simulink model "EV6_LUT_FourWheel_EV6Battery77p4kWh_PowerCorrected"  (R2024a)
settings: Solver=ode4  StartTime=0  StopTime=60  FixedStep=0.001  RelTol=1e-3
PreLoadFcn:
  | VSS_BICYCLE=Simulink.Variant('Dual=0');
  | VSS_DUAL=Simulink.Variant('Dual=1');
  | Dual=1;
  | load('DriveCycle2.mat')
PostLoadFcn:
  | if any(exist('dsrtsu_mdlpostloadfcn', 'file') ~= 0), dsrtsu_mdlpostloadfcn('Execute', bdroot); end
InitFcn:
  | , if any(exist('rtifpga_mdlclblib', 'file') ~= 0), rtifpga_mdlclblib('Init', bdroot); end,
  | , if any(exist('dsmpb_private', 'file') ~= 0), dsmpb_private('dsmpb_mdlclblib', 'Init', bdroot); end,
  | load('DriveCycle2.mat')
model workspace (MAT data in the model file):
  DiffRatio = 10.65
  EV6_2023_BattBranchCapacity_Ah = 55.5236728838
  EV6_2023_BattEnergy_kWh = 77.4
  EV6_2023_BattNominalVoltage_V = 697
  EV6_2023_BattNumCellsParallel = 2
  EV6_2023_BattNumCellsSeries = 192
  EV6_2023_BattOpenVoltCapBpts = [0 0.1 0.2 0.3 0.4 0.5 0.6 0.7 0.8 0.9 1]
  EV6_2023_BattOpenVoltTbl = [2.96762142548 3.40364281191 3.47417488548 3.54470541822 3.61523441014 3.68576186124 3.75628777151 3.82681214095 3.94527005036 4.07101207308 4.2120755254]
  EV6_2023_BattPackCapacity_Ah = 111.047345768
  EV6_2023_BattResistSocBpts = [0 0.2 0.4 0.6 0.8 1]
  EV6_2023_BattResistTbl = [0.0163620057716 0.0118174152018 0.00807187352333 0.00375663957972 0.00266904525531 0.00103635901355 0.0019014404175 0.0172368903217 0.0121226074867 0.00758541551769 0.00474065349228 0.00337561163613 ... (42 elements, 7x6)]
  EV6_2023_BattResistTempBpts = [243.1 253.1 263.1 273.1 283.1 298.1 313.1]
  EV6_2023_InitialPackOCV_V = 726.471714233
  EV6_2023_InitialSOC = 0.638878863672
  EV6_BattCellCapacity_Ah = 60.3
  EV6_BattInitialSOC = 0.638878863672
  EV6_BattOCV_Cell_V = [2.96762142548 3.40364281191 3.47417488548 3.54470541822 3.61523441014 3.68576186124 3.75628777151 3.82681214095 3.94527005036 4.07101207308 4.2120755254]
  EV6_BattOCV_SOC = [0 0.1 0.2 0.3 0.4 0.5 0.6 0.7 0.8 0.9 1]
  EV6_BattPackCapacity_Ah = 120.6
  EV6_BattParallelCells = 2
  EV6_BattResistanceSOC = [0 0.2 0.4 0.6 0.8 1]
  EV6_BattResistanceTable_Ohm = [0.0163620057716 0.0118174152018 0.00807187352333 0.00375663957972 0.00266904525531 0.00103635901355 0.0019014404175 0.0172368903217 0.0121226074867 0.00758541551769 0.00474065349228 0.00337561163613 ... (42 elements, 7x6)]
  EV6_BattResistanceTemp_K = [243.1 253.1 263.1 273.1 283.1 298.1 313.1]
  EV6_BattSeriesCells = 192
  EV6_FinalDriveRatio = 10.65
  EV6_TargetPackResistance_Ohm = 0.132763804608
  Gas = 0.383333333333
undefined symbols (not defined in the file): accel_bp_mps2, AccelCmd, ActTqLF_Nm_, ActTqLR_Nm_, ActTqRF_Nm_, ActTqRR_Nm_, BattChargeLimitMaxPwr, BattChargeLimitSocBpts, BattChargeLimitTbl, BattDischargeLimitSocBpts, BattDischargeLimitTbl, BattDischargeMaxPwr, BrakeMaxPrs, BrakeMaxTrq, ChassisDistCg2FrontAxle, ChassisDistCg2RearAxle, ChassisVehMass, CltchCmd, CoastDown, DecelCmd, DiscIntNeverNeededParam, EnvGravCnst, EnvPrs, EnvTemp, EV6_RegenTorqueGain, EV6_TractionTorqueGain, front_share_regen_3d, front_share_traction_3d, FuelSpecificGrav, GearCmd, h, InitStates, lgSw, limitedMCT, MCT, MtrEffSpdBpts, MtrEffTbl, MtrEffTrqBpts, MtrPwrMax, MtrTrqMax, out_1, pMCT, RealSimPara, Ref_speed, Ref_time, regen_torque_bp_Nm, speed_bp_kph, SteeringCmd, SupvsryCtrlRegenBrkCutOffTbl, SupvsryCtrlRegenSpdBpts, TestScnrioCycleNum, traction_torque_bp_Nm, US06, VEH
libraries: VSIGenLib x65, simulink x54, etargetslib x38, dsmpblib x24, vehdynlibtire x12, autolibshared x11, vehdynlibsuspension x7, vehdynlibtirecommon x7, autolibpowerinfoutils x6, autolibutils x5, autolibsharedcoupling x4, autolibmappedmotor x4
(part 3 of 19)

== system EV6_LUT_FourWheel_EV6Battery77p4kWh_PowerCorrected/RealSim1/ToRealSim/RealSim CreatBus ==
  In : Inport
  speedDesired : Inport  Port=2
  color : Inport  Port=3
  accelerationDesired : Inport  Port=4
  activeLaneChange : Inport  Port=5
  Bus Creator2 : BusCreator  Inputs=36  OutDataTypeStr=Bus: VehDataBus
  Bus Selector1 : BusSelector  OutputSignals=id,idLength,type,typeLength,vehicleClass,vehicleClassLength,speed,acceleration,positionX,positionY,positionZ,heading,color,linkId,linkIdLength,laneId,distanceTravel,speedDesired,accelerationDesired,hasPrecedingVehicle,precedingVehicleId,precedingVehicleIdLength,precedingVehicleDistance,precedingVehicleSpeed,signalLightId,signalLightIdLength,signalLightHeadId,signalLightDistance,signalLightColor,speedLimit,speedLimitNext,speedLimitChangeDistance,linkIdNext,linkIdNextLength,grade,activeLaneChange
  Terminator{4..7} (4 alike) : Terminator
  rgba2uint : Subsystem
  Out : Outport
  wires:
  Bus Creator2/1 -> Out/1
  rgba2uint/1(Out1) -> Bus Creator2/13  "color"
  color/1 -> rgba2uint/1(In1)  "color"
  accelerationDesired/1 -> Bus Creator2/19  "accelerationDesired"
  speedDesired/1 -> Bus Creator2/18  "speedDesired"
  activeLaneChange/1 -> Bus Creator2/36  "activeLaneChange"
  Bus Selector1/36 -> Terminator7/1  "<activeLaneChange>"
  Bus Selector1/35 -> Bus Creator2/35  "<grade>"
  Bus Selector1/34 -> Bus Creator2/34  "<linkIdNextLength>"
  Bus Selector1/33 -> Bus Creator2/33  "<linkIdNext>"
  Bus Selector1/32 -> Bus Creator2/32  "<speedLimitChangeDistance>"
  Bus Selector1/31 -> Bus Creator2/31  "<speedLimitNext>"
  Bus Selector1/30 -> Bus Creator2/30  "<speedLimit>"
  Bus Selector1/29 -> Bus Creator2/29  "<signalLightColor>"
  Bus Selector1/28 -> Bus Creator2/28  "<signalLightDistance>"
  Bus Selector1/27 -> Bus Creator2/27  "<signalLightHeadId>"
  Bus Selector1/26 -> Bus Creator2/26  "<signalLightIdLength>"
  Bus Selector1/25 -> Bus Creator2/25  "<signalLightId>"
  Bus Selector1/24 -> Bus Creator2/24  "<precedingVehicleSpeed>"
  Bus Selector1/23 -> Bus Creator2/23  "<precedingVehicleDistance>"
  Bus Selector1/22 -> Bus Creator2/22  "<precedingVehicleIdLength>"
  Bus Selector1/21 -> Bus Creator2/21  "<precedingVehicleId>"
  Bus Selector1/20 -> Bus Creator2/20  "<hasPrecedingVehicle>"
  Bus Selector1/19 -> Terminator6/1  "<accelerationDesired>"
  Bus Selector1/18 -> Terminator4/1  "<speedDesired>"
  Bus Selector1/17 -> Bus Creator2/17  "<distanceTravel>"
  Bus Selector1/16 -> Bus Creator2/16  "<laneId>"
  Bus Selector1/15 -> Bus Creator2/15  "<linkIdLength>"
  Bus Selector1/14 -> Bus Creator2/14  "<linkId>"
  Bus Selector1/13 -> Terminator5/1  "<color>"
  Bus Selector1/12 -> Bus Creator2/12  "<heading>"
  Bus Selector1/11 -> Bus Creator2/11  "<positionZ>"
  Bus Selector1/10 -> Bus Creator2/10  "<positionY>"
  Bus Selector1/9 -> Bus Creator2/9  "<positionX>"
  Bus Selector1/8 -> Bus Creator2/8  "<acceleration>"
  Bus Selector1/7 -> Bus Creator2/7  "<speed>"
  Bus Selector1/6 -> Bus Creator2/6  "<vehicleClassLength>"
  Bus Selector1/5 -> Bus Creator2/5  "<vehicleClass>"
  Bus Selector1/4 -> Bus Creator2/4  "<typeLength>"
  Bus Selector1/3 -> Bus Creator2/3  "<type>"
  Bus Selector1/2 -> Bus Creator2/2  "<idLength>"
  Bus Selector1/1 -> Bus Creator2/1  "<id>"
  In/1 -> Bus Selector1/1

== system EV6_LUT_FourWheel_EV6Battery77p4kWh_PowerCorrected/RealSim2/ToRealSim/RealSim CreatBus ==
  In : Inport
  speedDesired : Inport  Port=2
  color : Inport  Port=3
  accelerationDesired : Inport  Port=4
  activeLaneChange : Inport  Port=5
  Bus Creator2 : BusCreator  Inputs=36  OutDataTypeStr=Bus: VehDataBus
  Bus Selector1 : BusSelector  OutputSignals=id,idLength,type,typeLength,vehicleClass,vehicleClassLength,speed,acceleration,positionX,positionY,positionZ,heading,color,linkId,linkIdLength,laneId,distanceTravel,speedDesired,accelerationDesired,hasPrecedingVehicle,precedingVehicleId,precedingVehicleIdLength,precedingVehicleDistance,precedingVehicleSpeed,signalLightId,signalLightIdLength,signalLightHeadId,signalLightDistance,signalLightColor,speedLimit,speedLimitNext,speedLimitChangeDistance,linkIdNext,linkIdNextLength,grade,activeLaneChange
  Terminator{4..7} (4 alike) : Terminator
  rgba2uint : Subsystem
  Out : Outport
  wires:
  Bus Creator2/1 -> Out/1
  rgba2uint/1(Out1) -> Bus Creator2/13  "color"
  color/1 -> rgba2uint/1(In1)  "color"
  accelerationDesired/1 -> Bus Creator2/19  "accelerationDesired"
  speedDesired/1 -> Bus Creator2/18  "speedDesired"
  activeLaneChange/1 -> Bus Creator2/36  "activeLaneChange"
  Bus Selector1/36 -> Terminator7/1  "<activeLaneChange>"
  Bus Selector1/35 -> Bus Creator2/35  "<grade>"
  Bus Selector1/34 -> Bus Creator2/34  "<linkIdNextLength>"
  Bus Selector1/33 -> Bus Creator2/33  "<linkIdNext>"
  Bus Selector1/32 -> Bus Creator2/32  "<speedLimitChangeDistance>"
  Bus Selector1/31 -> Bus Creator2/31  "<speedLimitNext>"
  Bus Selector1/30 -> Bus Creator2/30  "<speedLimit>"
  Bus Selector1/29 -> Bus Creator2/29  "<signalLightColor>"
  Bus Selector1/28 -> Bus Creator2/28  "<signalLightDistance>"
  Bus Selector1/27 -> Bus Creator2/27  "<signalLightHeadId>"
  Bus Selector1/26 -> Bus Creator2/26  "<signalLightIdLength>"
  Bus Selector1/25 -> Bus Creator2/25  "<signalLightId>"
  Bus Selector1/24 -> Bus Creator2/24  "<precedingVehicleSpeed>"
  Bus Selector1/23 -> Bus Creator2/23  "<precedingVehicleDistance>"
  Bus Selector1/22 -> Bus Creator2/22  "<precedingVehicleIdLength>"
  Bus Selector1/21 -> Bus Creator2/21  "<precedingVehicleId>"
  Bus Selector1/20 -> Bus Creator2/20  "<hasPrecedingVehicle>"
  Bus Selector1/19 -> Terminator6/1  "<accelerationDesired>"
  Bus Selector1/18 -> Terminator4/1  "<speedDesired>"
  Bus Selector1/17 -> Bus Creator2/17  "<distanceTravel>"
  Bus Selector1/16 -> Bus Creator2/16  "<laneId>"
  Bus Selector1/15 -> Bus Creator2/15  "<linkIdLength>"
  Bus Selector1/14 -> Bus Creator2/14  "<linkId>"
  Bus Selector1/13 -> Terminator5/1  "<color>"
  Bus Selector1/12 -> Bus Creator2/12  "<heading>"
  Bus Selector1/11 -> Bus Creator2/11  "<positionZ>"
  Bus Selector1/10 -> Bus Creator2/10  "<positionY>"
  Bus Selector1/9 -> Bus Creator2/9  "<positionX>"
  Bus Selector1/8 -> Bus Creator2/8  "<acceleration>"
  Bus Selector1/7 -> Bus Creator2/7  "<speed>"
  Bus Selector1/6 -> Bus Creator2/6  "<vehicleClassLength>"
  Bus Selector1/5 -> Bus Creator2/5  "<vehicleClass>"
  Bus Selector1/4 -> Bus Creator2/4  "<typeLength>"
  Bus Selector1/3 -> Bus Creator2/3  "<type>"
  Bus Selector1/2 -> Bus Creator2/2  "<idLength>"
  Bus Selector1/1 -> Bus Creator2/1  "<id>"
  In/1 -> Bus Selector1/1

== system EV6_LUT_FourWheel_EV6Battery77p4kWh_PowerCorrected/Vehicle Under Test1/Environment/Ground Feedback ==
  note: 1) Add Subsystem or Model blocks as valid variant choices.
      | 2) You cannot connect blocks at this level. At simulation, connectivity is automatically
      | determined, based on the active variant and port name matching.
  Friction : Inport
  Ground Z Level : Inport  Port=2
  3D Engine : Subsystem  VariantControl=1
  Constant : Subsystem  VariantControl=0
  Ground : Outport  VectorParamsAs1DForOutWhenUnconnected=off

== system EV6_LUT_FourWheel_EV6Battery77p4kWh_PowerCorrected/Vehicle Under Test1/Environment/Subsystem ==
  Grade : Inport
  Constant : Constant  Value=EnvPrs
  Constant1 : Constant  Value=EnvTemp
  Constant2 : Constant  Value=0
  Constant3 : Constant  Value=0
  Constant4 : Constant  Value=0
  Signal Specification : SignalSpecification  Unit=Pa
  Signal Specification1 : SignalSpecification  Unit=K
  Signal Specification2 : SignalSpecification  Unit=rad
  Signal Specification3 : SignalSpecification  Unit=m/s
  Signal Specification4 : SignalSpecification  Unit=m/s
  Signal Specification5 : SignalSpecification  Unit=m/s
  Vector Concatenate : Concatenate  NumInputs=3
  EnvPrs : Outport
  EnvTemp : Outport  Port=2
  WindVel : Outport  Port=3
  RoadGrade : Outport  Port=4
  wires:
  Signal Specification5/1 -> Vector Concatenate/3  "WindZ"
  Signal Specification4/1 -> Vector Concatenate/2  "WindY"
  Constant4/1 -> Signal Specification5/1
  Constant3/1 -> Signal Specification4/1
  Signal Specification3/1 -> Vector Concatenate/1  "WindX"
  Vector Concatenate/1 -> WindVel/1
  Signal Specification2/1 -> RoadGrade/1
  Signal Specification1/1 -> EnvTemp/1
  Signal Specification/1 -> EnvPrs/1
  Grade/1 -> Signal Specification2/1
  Constant1/1 -> Signal Specification1/1
  Constant2/1 -> Signal Specification3/1
  Constant/1 -> Signal Specification/1

== system EV6_LUT_FourWheel_EV6Battery77p4kWh_PowerCorrected/Vehicle Under Test1/Environment/Subsystem1 ==
  EnvPrs : Inport
  EnvTemp : Inport  Port=2
  WindVel : Inport  Port=3
  RoadGrade : Inport  Port=4
  GroundBus : Inport  Port=5
  Bus Creator : BusCreator  Inputs=5
  Env : Outport
  wires:
  GroundBus/1 -> Bus Creator/5  "GndBus"
  RoadGrade/1 -> Bus Creator/4  "RoadGrade"
  WindVel/1 -> Bus Creator/3  "WindVel"
  Bus Creator/1 -> Env/1  "Env"
  EnvTemp/1 -> Bus Creator/2  "EnvTemp"
  EnvPrs/1 -> Bus Creator/1  "EnvPrs"

== system EV6_LUT_FourWheel_EV6Battery77p4kWh_PowerCorrected/Vehicle Under Test1/Monitor/Calculate Fuel MPG ==
  Monitor : Inport
  Bus Selector : BusSelector  OutputSignals=Veh.Chassis.VehDist,Veh.Batt.EngPlant.FuellMassFlw
  Constant : Constant  Value=FuelSpecificGrav
  Density of Water : Gain  Gain=997
  Divide : Product  Inputs=*/
  Divide1 : Product  Inputs=*/
  Integrator : Integrator
  Saturation : Saturate  UpperLimit=inf  LowerLimit=1e-7
  Signal Specification : SignalSpecification  Unit=mi
  Signal Specification1 : SignalSpecification  Unit=m^3
  Signal Specification2 : SignalSpecification  Unit=gal
  Unit Conversion : UnitConversion
  Unit Conversion1 : UnitConversion
  FuelEconMPG : Outport
  wires:
  Signal Specification/1 -> Divide1/1  "VehDistMiles"
  Monitor/1 -> Bus Selector/1
  Signal Specification1/1 -> Unit Conversion1/1
  Constant/1 -> Density of Water/1
  Saturation/1 -> Divide1/2  "FuelVolume"
  Density of Water/1 -> Divide/2
  Integrator/1 -> Divide/1  "FuelMass"
  Bus Selector/2 -> Integrator/1  "<FuellMassFlw>"
  Bus Selector/1 -> Unit Conversion/1  "<VehDist>"
  Unit Conversion/1 -> Signal Specification/1
  Signal Specification2/1 -> Saturation/1
  Unit Conversion1/1 -> Signal Specification2/1
  Divide/1 -> Signal Specification1/1
  Divide1/1 -> FuelEconMPG/1  "FuelEconMPG"

== system EV6_LUT_FourWheel_EV6Battery77p4kWh_PowerCorrected/Vehicle Under Test1/Monitor/Calculate Powertrain Energy ==
  Monitor : Inport
  Bus Selector2 : BusSelector  OutputSignals=Veh.Diff.PwrInfo.PwrTrnsfrd.PwrTrnsfrd.PwrDriveshft
  Integrator : Integrator
  Signal Specification : SignalSpecification  Unit=J
  Signal Specification1 : SignalSpecification  Unit=kW*h
  Unit Conversion : UnitConversion
  TransEnrgyOutkWh : Outport
  wires:
  Bus Selector2/1 -> Integrator/1  "<PwrDriveshft>"
  Monitor/1 -> Bus Selector2/1
  Signal Specification1/1 -> TransEnrgyOutkWh/1
  Signal Specification/1 -> Unit Conversion/1
  Integrator/1 -> Signal Specification/1  "EnrgyTrans"
  Unit Conversion/1 -> Signal Specification1/1

== system EV6_LUT_FourWheel_EV6Battery77p4kWh_PowerCorrected/Vehicle Under Test1/Vehicle/Actuation and Outputs ==
  note: Driver Commands are [0,100] for both pedal and brake
  Driver Commands : Inport
  CarlaGBS : Inport  Port=2
  APP : Constant  Value=0
  AR_limit : Saturate  UpperLimit=65  LowerLimit=0
  BR_command_0to100 : Constant  Value=0
  BR_limit : Saturate  UpperLimit=70  LowerLimit=0
  Bus Creator : BusCreator  Inputs=2
  Bus Selector1 : BusSelector  OutputSignals=AccelPedalCmd
  Bus Selector3 : BusSelector  OutputSignals=BrakePedalCmd
  Constant : Constant  Value=0
  Constant1 : Constant  Value=0
  Demux : Demux  Outputs=3
  Gain : Gain  Gain=100
  Gain1 : Gain  Gain=100
  MOOG Brake Actuator : Subsystem
  Min threshold for Brake switch : Constant  Value=0
  Multiport Switch1 : MultiPortSwitch  Inputs=4  SaturateOnIntegerOverflow=off  InputSameDT=off
  Multiport Switch2 : MultiPortSwitch  Inputs=4  SaturateOnIntegerOverflow=off  InputSameDT=off
  Pedal Robot Control Selection : Constant  Value=2
  Relational Operator : RelationalOperator  Operator=>  OutDataTypeStr=boolean  InputSameDT=off
  Scope1 : Scope  NumInputPorts=2
  Vehicle Accel Pedal Voltage Output : Subsystem
  bped2br_N : Lookup_n-D  NumberOfTableDimensions=1  BreakpointsForDimension1=[0 0.1 0.2 100]  Table=[0 0 25 100]  InternalRulePriority=Speed  RndMeth=Simplest
  BrakeSwitch : Outport  VectorParamsAs1DForOutWhenUnconnected=off
  CAVE_Driver : Outport  Port=2
  tag scope: BrakeDriver=global, CarlaSteer=global, GasDriver=global
  wires:
  [BrakeDriver] -> Scope1/2
  [GasDriver] -> Scope1/1
  Demux/3 -> [CarlaSteer]
  Gain1/1 -> Multiport Switch2/4
  Gain/1 -> Multiport Switch1/4
  CarlaGBS/1 -> Demux/1
  Demux/2 -> Gain1/1
  Demux/1 -> Gain/1
  BR_limit/1 -> bped2br_N/1, Relational Operator/1, Bus Creator/2, [BrakeDriver]  "BrakePedalCmd_pct"
  AR_limit/1 -> Vehicle Accel Pedal Voltage Output/1(APP_pct), Bus Creator/1, [GasDriver]  "AccelPedalCmd_pct"
  Bus Creator/1 -> CAVE_Driver/1
  Constant1/1 -> Multiport Switch2/5
  Constant/1 -> Multiport Switch1/5
  Relational Operator/1 -> BrakeSwitch/1  "BrakeSwitch"
  Min threshold for Brake switch/1 -> Relational Operator/2
  bped2br_N/1 -> MOOG Brake Actuator/1(Brake Pedal command [%])  "BrakeActuatorCmd_N"
  Bus Selector3/1 -> Multiport Switch2/3  "<BrakePedalCmd>"
  BR_command_0to100/1 -> Multiport Switch2/2
  Pedal Robot Control Selection/1 -> Multiport Switch2/1, Multiport Switch1/1
  Driver Commands/1 -> Bus Selector1/1, Bus Selector3/1
  Multiport Switch2/1 -> BR_limit/1
  Bus Selector1/1 -> Multiport Switch1/3  "<AccelPedalCmd>"
  APP/1 -> Multiport Switch1/2
  Multiport Switch1/1 -> AR_limit/1

== system EV6_LUT_FourWheel_EV6Battery77p4kWh_PowerCorrected/Vehicle Under Test1/Vehicle/Battery ==
  Battery : Subsystem
  Subsystem1 : Subsystem
      mask Display: disp('')
  BattOut : PMIOPort  Side=Right
  BattOut1 : PMIOPort  Port=2  Side=Right
  Batt : Outport
  wires:
  Subsystem1/1(Batt) -> Batt/1
  Battery/3(BattVolt) -> Subsystem1/3(BattVolt)
  Battery/2(BattCurr) -> Subsystem1/2(BattCurr)
  Battery/1(BattSoc) -> Subsystem1/1(BattSoc)
  connections:
  BattOut/RConn1 -- Battery/RConn1
  Battery/RConn2 -- BattOut1/RConn1

== system EV6_LUT_FourWheel_EV6Battery77p4kWh_PowerCorrected/Vehicle Under Test1/Vehicle/Driver and Drive Cycle ==
  Veh speed feedback [kph] : Inport
  Veh speed cycle trigger : Inport  Port=2
  SUMO Veh speed Cmd Level : Inport  Port=3
  CarlaRef : Inport  Port=4
  1-D Lookup Table : Lookup_n-D  NumberOfTableDimensions=1  BreakpointsForDimension1=Ref_time  Table=Ref_speed  InternalRulePriority=Speed  RndMeth=Simplest
  Add : Sum
  Add1 : Sum  Inputs=+-
  Add2 : Sum
  Clock : Clock
  Clock1 : Clock
  CoastDown : Lookup_n-D  Commented=on  NumberOfTableDimensions=1  BreakpointsForDimension1=CoastDown.Time  Table=CoastDown.Speed  InternalRulePriority=Speed  RndMeth=Simplest
  Constant : Constant  Value=0
  Data Type Conversion11 : DataTypeConversion  OutDataTypeStr=double  SaturateOnIntegerOverflow=off  RndMeth=Floor  LockScale=on
  Demux : Demux  Outputs=3
  DriveCycleSelect : Constant  Commented=on
  Driver and PI with FF Control : Subsystem
  Gain : Gain  Gain=1/1.609
  Gain1 : Gain  Gain=1/1.609
  Gain2 : Gain  Gain=3.6
  Gain3 : Gain  Gain=3.6
  Get Cycle Clock Time : Subsystem
  MCT : Lookup_n-D  Commented=on  NumberOfTableDimensions=1  BreakpointsForDimension1=MCT.Time  Table=MCT.Speed  InternalRulePriority=Speed  RndMeth=Simplest
  ManSpd : Constant  Value=0
  ManSpdSel1 : Constant  Value=2
  Memory4 : Memory
  Multiport Switch : MultiPortSwitch  Commented=on  Inputs=5  SaturateOnIntegerOverflow=off  InputSameDT=off
  Multiport Switch1 : MultiPortSwitch  Inputs=4  SaturateOnIntegerOverflow=off  InputSameDT=off
  Rate Limiter : RateLimiter  RisingSlewLimit=5  FallingSlewLimit=-5  SampleTimeMode=inherited
  Scope : Scope  NumInputPorts=2
  Switch1 : Switch  Threshold=3  SaturateOnIntegerOverflow=off  InputSameDT=off
  Terminator{,1..3} (4 alike) : Terminator
  Terminator4 : Terminator  Commented=on
  US06 : Lookup_n-D  Commented=on  NumberOfTableDimensions=1  BreakpointsForDimension1=US06.Time  Table=US06.Speed  InternalRulePriority=Speed  RndMeth=Simplest
  US1 : Lookup_n-D  NumberOfTableDimensions=1  BreakpointsForDimension1=US06.Time  Table=US06.Speed  InternalRulePriority=Speed  RndMeth=Simplest
  driver look ahead seconds : Constant  Value=0.5
  limitedMCT : Lookup_n-D  Commented=on  NumberOfTableDimensions=1  BreakpointsForDimension1=limitedMCT.Time  Table=limitedMCT.Speed  InternalRulePriority=Speed  RndMeth=Simplest
  pMCT : Lookup_n-D  Commented=on  NumberOfTableDimensions=1  BreakpointsForDimension1=pMCT.Time  Table=pMCT.Speed  InternalRulePriority=Speed  RndMeth=Simplest
  DriverBus : Outport
  ManSpdSel : Outport  Port=2
  wires:
  US1/1 -> Rate Limiter/1
  Clock/1 -> Switch1/3
  Add2/1 -> Gain3/1
  Gain3/1 -> Multiport Switch1/4
  Memory4/1 -> Switch1/1
  Switch1/1 -> Memory4/1, Add1/2
  SUMO Veh speed Cmd Level/1 -> Add2/2
  Add1/1 -> 1-D Lookup Table/1  "tCycle"
  1-D Lookup Table/1 -> Add2/1
  ManSpdSel1/1 -> ManSpdSel/1, Multiport Switch1/1, Switch1/2
  Clock1/1 -> Add1/1, US1/1
  Constant/1 -> Multiport Switch1/5
  Demux/3 -> Terminator3/1
  Demux/2 -> Terminator2/1
  Demux/1 -> Gain2/1
  CarlaRef/1 -> Demux/1
  Gain2/1 -> Multiport Switch1/3
  Multiport Switch/1 -> Terminator4/1
  Rate Limiter/1 -> Multiport Switch1/2
  Multiport Switch1/1 -> Driver and PI with FF Control/2(Vehicle_SpdDmd_kph), Gain1/1, Scope/2  "RefSpd [km/hr]"
  Gain1/1 -> Terminator1/1  "Vehicle_SpdDmd_mph"
  Gain/1 -> Terminator/1  "Vehicle_Spd_mph"
  Veh speed feedback [kph]/1 -> [VehSpdKph]
  limitedMCT/1 -> Multiport Switch/6
  driver look ahead seconds/1 -> Add/1
  Get Cycle Clock Time/1(tCycle) -> Add/2
  Data Type Conversion11/1 -> Driver and PI with FF Control/1(Vehicle_Spd_kph), Scope/1, Gain/1  "Vehicle_Spd_kph"
  Driver and PI with FF Control/1(DriverBus) -> DriverBus/1
  [VehSpdKph] -> Data Type Conversion11/1
  DriveCycleSelect/1 -> Multiport Switch/1
  pMCT/1 -> Multiport Switch/3
  CoastDown/1 -> Multiport Switch/2
  Add/1 -> US06/1, MCT/1, limitedMCT/1, pMCT/1, CoastDown/1
  US06/1 -> Multiport Switch/4
  MCT/1 -> Multiport Switch/5
  Veh speed cycle trigger/1 -> Get Cycle Clock Time/1(Cycle Trigger)

== system EV6_LUT_FourWheel_EV6Battery77p4kWh_PowerCorrected/Vehicle Under Test1/Vehicle/From CAN ==
  BrakeSwitch : Inport
  Brake switch ource selection : Constant  Value=2
  Bus Creator1 : BusCreator  Inputs=2
  Demux : Demux  Outputs=1
  Ground : Ground
  Ground1 : Ground
  Multiport Switch1 : MultiPortSwitch  Inputs=2  SaturateOnIntegerOverflow=off  InputSameDT=off
  IO_Out : Outport
  wires:
  BrakeSwitch/1 -> Multiport Switch1/3
  Ground1/1 -> Multiport Switch1/2  "Brake switch from CAN"
  Brake switch ource selection/1 -> Multiport Switch1/1
  Ground/1 -> Demux/1
  Demux/1 -> Bus Creator1/1  "STEERING_ANGLE_DEG_CAN"
  Multiport Switch1/1 -> Bus Creator1/2  "BRAKE_LAMP_BOOL_CAN"
  Bus Creator1/1 -> IO_Out/1  "IO_Out"

== system EV6_LUT_FourWheel_EV6Battery77p4kWh_PowerCorrected/Vehicle Under Test1/Vehicle/Front Wheel Drive ==
  DrvShfTrq : Inport
  Omega : Inport  Port=2
  Ideal Diff : Subsystem  VariantControl=0
  Ideal Diff AWD : Subsystem  VariantControl=Choice
  Real Diff : Subsystem  VariantControl=1
  Diff : Outport  VectorParamsAs1DForOutWhenUnconnected=off
  AxlTrq : Outport  Port=2  VectorParamsAs1DForOutWhenUnconnected=off
  PropShaftSpd : Outport  Port=3  VectorParamsAs1DForOutWhenUnconnected=off
  PropShaftSpd1 : Outport  Port=4
